simulink model "s_b16a4x32kf"  (R2018a)
settings: Solver=VariableStepDiscrete  StartTime=0.0  StopTime=1000  RelTol=1e-3
undefined symbols (not defined in the file): fft_stages, n_bits_ants, n_bits_xengs
libraries: xbsIndex_r4 x23740, casper_library_misc x48, casper_library_delays x8, xps_library x4, casper_library_scopes x1
(part 126 of 219)

== system s_b16a4x32kf/sys3/xeng/baseline_tap2/dual_pol_cmac/cmac ==
  a+bi : Inport
  c+di : Inport  Port=2
  acc_in : Inport  Port=3
  sync : Inport  Port=4
  valid_in : Inport  Port=5
  Constant1 : xbsIndex_r4/Constant  const=0  gui_display_data_type=Fixed-point  arith_type=Unsigned  n_bits=bit_growth  bin_pt=0  preci_type=Single  exp_width=8  frac_width=24  explicit_period=on  period=1  equ=P=C  opselect=C  inp2=PCIN>>17  opr=+  inp1=P  carry=CIN  dbl_ovrd=off  block_type=constant
      settings: block_version=9.2.01
  Constant2 : xbsIndex_r4/Constant  const=0  gui_display_data_type=Fixed-point  arith_type=Unsigned  n_bits=1  bin_pt=0  preci_type=Single  exp_width=8  frac_width=24  explicit_period=off  period=1  equ=P=C  opselect=C  inp2=PCIN>>17  opr=+  inp1=P  carry=CIN  dbl_ovrd=off  block_type=constant
      settings: block_version=9.2.01
  Counter : xbsIndex_r4/Counter  cnt_type=Count Limited  cnt_to=acc_len - 1  operation=Up  start_count=0  cnt_by_val=1  arith_type=Unsigned  n_bits=bit_growth  bin_pt=0  load_pin=off  rst=on  en=off  explicit_period=off  period=1  use_behavioral_HDL=off  implementation=Fabric  use_rpm=on  dbl_ovrd=off  block_type=counter
      settings: xl_area=[0, 0, 0, 0, 0, 0, 0]  block_version=9.2.01
  Delay : xbsIndex_r4/Delay  rst=off  infoeditControl=Selection of Reset will increase slice count due to use of real FFs and instead of SRLs  en=off  latency=add_latency + mult_latency - 1  reg_retiming=on  dbl_ovrd=off  block_type=delay
      settings: xl_area=[0, 0, 0, 0, 0, 0, 0]  block_version=9.2.01
  Relational : xbsIndex_r4/Relational  mode=a=b  op_type=Bool  en=off  latency=1  dbl_ovrd=off  block_type=relational
      settings: xl_area=[0, 0, 0, 0, 0, 0, 0]  block_version=9.2.01
  Terminator : Terminator
  acc : Subsystem
  acc1 : Subsystem
  c_to_ri1 : Subsystem
  c_to_ri2 : Subsystem
  cmult* : Subsystem  AncestorBlock=casper_library_multipliers/cmult  mask(cmult){n_bits_a=8, bin_pt_a=7, n_bits_b=8, bin_pt_b=7, n_bits_ab=25, bin_pt_ab=14, quantization=Truncate, overflow=Wrap, in_latency=0, mult_latency=4, add_latency=3, conv_latency=0, conjugated=on, async=off, pipelined_enable=on, multiplier_implementation=embedded multiplier core}
      mask prompts: n_bits_a "Number of Bits 'a'"; bin_pt_a "Binary Point 'a'"; n_bits_b "Number of Bits 'b'"; bin_pt_b "Binary Point 'b'"; n_bits_ab "Number of Bits 'ab'"; bin_pt_ab "Binary Point 'ab'"; in_latency "Input latency"; mult_latency "Multiplier Latency"; add_latency "Adder Latency"; conv_latency "Convert latency"; conjugated "Conjugate"; async "asynchronous operation"; pipelined_enable "enable pipeline"; multiplier_implementation "Multiplier implementation"
      mask help:
      | Multiplies two complex numbers using 4 multipliers and 2 adders.
      | Conjugation is optional.
      mask init: same as s_b16a4x32kf/sys0/xeng/auto_tap/dual_pol_cmac/cmac/cmult*
      settings: AttributesFormatString=|
      | 8_7 * 8_7 ==> 25_14
      | Truncate, Wrap
      | Latency=0
      mask TypeOptions quantization: Truncate | Round  (unbiased: +/- Inf) | Round  (unbiased: Even Values)
      mask TypeOptions overflow: Wrap | Saturate | Flag as error
      mask TypeOptions multiplier_implementation: behavioral HDL | standard core | embedded multiplier core
  ri_to_c : Subsystem
  acc_out : Outport
  valid_out : Outport  Port=2
  wires:
  cmult*/1(ab) -> c_to_ri1/1(In1)
  valid_in/1 -> acc1/4(valid_in)
  acc1/2(valid_out) -> valid_out/1
  acc/2(valid_out) -> Terminator/1
  Constant2/1 -> acc/4(valid_in)
  Delay/1 -> Counter/1
  sync/1 -> Delay/1
  Constant1/1 -> Relational/2
  Counter/1 -> Relational/1
  Relational/1 -> acc1/1(rst), acc/1(rst)
  c_to_ri2/2(Out2) -> acc1/3(acc_in)
  ri_to_c/1(Out1) -> acc_out/1
  acc1/1(acc_out) -> ri_to_c/2(In2)
  acc_in/1 -> c_to_ri2/1(In1)
  c+di/1 -> cmult*/2(b)
  a+bi/1 -> cmult*/1(a)
  c_to_ri1/1(Out1) -> acc/2(din)  "auto_real"
  c_to_ri1/2(Out2) -> acc1/2(din)
  acc/1(acc_out) -> ri_to_c/1(In1)
  c_to_ri2/1(Out1) -> acc/3(acc_in)

== system s_b16a4x32kf/sys3/xeng/baseline_tap2/dual_pol_cmac/cmac1 ==
  a+bi : Inport
  c+di : Inport  Port=2
  acc_in : Inport  Port=3
  sync : Inport  Port=4
  valid_in : Inport  Port=5
  Constant1 : xbsIndex_r4/Constant  const=0  gui_display_data_type=Fixed-point  arith_type=Unsigned  n_bits=bit_growth  bin_pt=0  preci_type=Single  exp_width=8  frac_width=24  explicit_period=on  period=1  equ=P=C  opselect=C  inp2=PCIN>>17  opr=+  inp1=P  carry=CIN  dbl_ovrd=off  block_type=constant
      settings: block_version=9.2.01
  Constant2 : xbsIndex_r4/Constant  const=0  gui_display_data_type=Fixed-point  arith_type=Unsigned  n_bits=1  bin_pt=0  preci_type=Single  exp_width=8  frac_width=24  explicit_period=off  period=1  equ=P=C  opselect=C  inp2=PCIN>>17  opr=+  inp1=P  carry=CIN  dbl_ovrd=off  block_type=constant
      settings: block_version=9.2.01
  Counter : xbsIndex_r4/Counter  cnt_type=Count Limited  cnt_to=acc_len - 1  operation=Up  start_count=0  cnt_by_val=1  arith_type=Unsigned  n_bits=bit_growth  bin_pt=0  load_pin=off  rst=on  en=off  explicit_period=off  period=1  use_behavioral_HDL=off  implementation=Fabric  use_rpm=on  dbl_ovrd=off  block_type=counter
      settings: xl_area=[0, 0, 0, 0, 0, 0, 0]  block_version=9.2.01
  Delay : xbsIndex_r4/Delay  rst=off  infoeditControl=Selection of Reset will increase slice count due to use of real FFs and instead of SRLs  en=off  latency=add_latency + mult_latency - 1  reg_retiming=on  dbl_ovrd=off  block_type=delay
      settings: xl_area=[0, 0, 0, 0, 0, 0, 0]  block_version=9.2.01
  Relational : xbsIndex_r4/Relational  mode=a=b  op_type=Bool  en=off  latency=1  dbl_ovrd=off  block_type=relational
      settings: xl_area=[0, 0, 0, 0, 0, 0, 0]  block_version=9.2.01
  Terminator : Terminator
  acc : Subsystem
  acc1 : Subsystem
  c_to_ri1 : Subsystem
  c_to_ri2 : Subsystem
  cmult* : Subsystem  AncestorBlock=casper_library_multipliers/cmult  mask(cmult){n_bits_a=8, bin_pt_a=7, n_bits_b=8, bin_pt_b=7, n_bits_ab=25, bin_pt_ab=14, quantization=Truncate, overflow=Wrap, in_latency=0, mult_latency=4, add_latency=3, conv_latency=0, conjugated=on, async=off, pipelined_enable=on, multiplier_implementation=embedded multiplier core}
      mask prompts: n_bits_a "Number of Bits 'a'"; bin_pt_a "Binary Point 'a'"; n_bits_b "Number of Bits 'b'"; bin_pt_b "Binary Point 'b'"; n_bits_ab "Number of Bits 'ab'"; bin_pt_ab "Binary Point 'ab'"; in_latency "Input latency"; mult_latency "Multiplier Latency"; add_latency "Adder Latency"; conv_latency "Convert latency"; conjugated "Conjugate"; async "asynchronous operation"; pipelined_enable "enable pipeline"; multiplier_implementation "Multiplier implementation"
      mask help:
      | Multiplies two complex numbers using 4 multipliers and 2 adders.
      | Conjugation is optional.
      mask init: same as s_b16a4x32kf/sys0/xeng/auto_tap/dual_pol_cmac/cmac/cmult*
      settings: AttributesFormatString=|
      | 8_7 * 8_7 ==> 25_14
      | Truncate, Wrap
      | Latency=0
      mask TypeOptions quantization: Truncate | Round  (unbiased: +/- Inf) | Round  (unbiased: Even Values)
      mask TypeOptions overflow: Wrap | Saturate | Flag as error
      mask TypeOptions multiplier_implementation: behavioral HDL | standard core | embedded multiplier core
  ri_to_c : Subsystem
  acc_out : Outport
  valid_out : Outport  Port=2
  wires:
  cmult*/1(ab) -> c_to_ri1/1(In1)
  valid_in/1 -> acc1/4(valid_in)
  acc1/2(valid_out) -> valid_out/1
  acc/2(valid_out) -> Terminator/1
  Constant2/1 -> acc/4(valid_in)
  Delay/1 -> Counter/1
  sync/1 -> Delay/1
  Constant1/1 -> Relational/2
  Counter/1 -> Relational/1
  Relational/1 -> acc1/1(rst), acc/1(rst)
  c_to_ri2/2(Out2) -> acc1/3(acc_in)
  ri_to_c/1(Out1) -> acc_out/1
  acc1/1(acc_out) -> ri_to_c/2(In2)
  acc_in/1 -> c_to_ri2/1(In1)
  c+di/1 -> cmult*/2(b)
  a+bi/1 -> cmult*/1(a)
  c_to_ri1/1(Out1) -> acc/2(din)  "auto_real"
  c_to_ri1/2(Out2) -> acc1/2(din)
  acc/1(acc_out) -> ri_to_c/1(In1)
  c_to_ri2/1(Out1) -> acc/3(acc_in)

== system s_b16a4x32kf/sys3/xeng/baseline_tap2/dual_pol_cmac/cmac2 ==
  a+bi : Inport
  c+di : Inport  Port=2
  acc_in : Inport  Port=3
  sync : Inport  Port=4
  valid_in : Inport  Port=5
  Constant1 : xbsIndex_r4/Constant  const=0  gui_display_data_type=Fixed-point  arith_type=Unsigned  n_bits=bit_growth  bin_pt=0  preci_type=Single  exp_width=8  frac_width=24  explicit_period=on  period=1  equ=P=C  opselect=C  inp2=PCIN>>17  opr=+  inp1=P  carry=CIN  dbl_ovrd=off  block_type=constant
      settings: block_version=9.2.01
  Constant2 : xbsIndex_r4/Constant  const=0  gui_display_data_type=Fixed-point  arith_type=Unsigned  n_bits=1  bin_pt=0  preci_type=Single  exp_width=8  frac_width=24  explicit_period=off  period=1  equ=P=C  opselect=C  inp2=PCIN>>17  opr=+  inp1=P  carry=CIN  dbl_ovrd=off  block_type=constant
      settings: block_version=9.2.01
  Counter : xbsIndex_r4/Counter  cnt_type=Count Limited  cnt_to=acc_len - 1  operation=Up  start_count=0  cnt_by_val=1  arith_type=Unsigned  n_bits=bit_growth  bin_pt=0  load_pin=off  rst=on  en=off  explicit_period=off  period=1  use_behavioral_HDL=off  implementation=Fabric  use_rpm=on  dbl_ovrd=off  block_type=counter
      settings: xl_area=[0, 0, 0, 0, 0, 0, 0]  block_version=9.2.01
  Delay : xbsIndex_r4/Delay  rst=off  infoeditControl=Selection of Reset will increase slice count due to use of real FFs and instead of SRLs  en=off  latency=add_latency + mult_latency - 1  reg_retiming=on  dbl_ovrd=off  block_type=delay
      settings: xl_area=[0, 0, 0, 0, 0, 0, 0]  block_version=9.2.01
  Relational : xbsIndex_r4/Relational  mode=a=b  op_type=Bool  en=off  latency=1  dbl_ovrd=off  block_type=relational
      settings: xl_area=[0, 0, 0, 0, 0, 0, 0]  block_version=9.2.01
  Terminator : Terminator
  acc : Subsystem
  acc1 : Subsystem
  c_to_ri1 : Subsystem
  c_to_ri2 : Subsystem
  cmult* : Subsystem  AncestorBlock=casper_library_multipliers/cmult  mask(cmult){n_bits_a=8, bin_pt_a=7, n_bits_b=8, bin_pt_b=7, n_bits_ab=25, bin_pt_ab=14, quantization=Truncate, overflow=Wrap, in_latency=0, mult_latency=4, add_latency=3, conv_latency=0, conjugated=on, async=off, pipelined_enable=on, multiplier_implementation=embedded multiplier core}
      mask prompts: n_bits_a "Number of Bits 'a'"; bin_pt_a "Binary Point 'a'"; n_bits_b "Number of Bits 'b'"; bin_pt_b "Binary Point 'b'"; n_bits_ab "Number of Bits 'ab'"; bin_pt_ab "Binary Point 'ab'"; in_latency "Input latency"; mult_latency "Multiplier Latency"; add_latency "Adder Latency"; conv_latency "Convert latency"; conjugated "Conjugate"; async "asynchronous operation"; pipelined_enable "enable pipeline"; multiplier_implementation "Multiplier implementation"
      mask help:
      | Multiplies two complex numbers using 4 multipliers and 2 adders.
      | Conjugation is optional.
      mask init: same as s_b16a4x32kf/sys0/xeng/auto_tap/dual_pol_cmac/cmac/cmult*
      settings: AttributesFormatString=|
      | 8_7 * 8_7 ==> 25_14
      | Truncate, Wrap
      | Latency=0
      mask TypeOptions quantization: Truncate | Round  (unbiased: +/- Inf) | Round  (unbiased: Even Values)
      mask TypeOptions overflow: Wrap | Saturate | Flag as error
      mask TypeOptions multiplier_implementation: behavioral HDL | standard core | embedded multiplier core
  ri_to_c : Subsystem
  acc_out : Outport
  valid_out : Outport  Port=2
  wires:
  cmult*/1(ab) -> c_to_ri1/1(In1)
  valid_in/1 -> acc1/4(valid_in)
  acc1/2(valid_out) -> valid_out/1
  acc/2(valid_out) -> Terminator/1
  Constant2/1 -> acc/4(valid_in)
  Delay/1 -> Counter/1
  sync/1 -> Delay/1
  Constant1/1 -> Relational/2
  Counter/1 -> Relational/1
  Relational/1 -> acc1/1(rst), acc/1(rst)
  c_to_ri2/2(Out2) -> acc1/3(acc_in)
  ri_to_c/1(Out1) -> acc_out/1
  acc1/1(acc_out) -> ri_to_c/2(In2)
  acc_in/1 -> c_to_ri2/1(In1)
  c+di/1 -> cmult*/2(b)
  a+bi/1 -> cmult*/1(a)
  c_to_ri1/1(Out1) -> acc/2(din)  "auto_real"
  c_to_ri1/2(Out2) -> acc1/2(din)
  acc/1(acc_out) -> ri_to_c/1(In1)
  c_to_ri2/1(Out1) -> acc/3(acc_in)

== system s_b16a4x32kf/sys3/xeng/baseline_tap2/dual_pol_cmac/cmac3 ==
  a+bi : Inport
  c+di : Inport  Port=2
  acc_in : Inport  Port=3
  sync : Inport  Port=4
  valid_in : Inport  Port=5
  Constant1 : xbsIndex_r4/Constant  const=0  gui_display_data_type=Fixed-point  arith_type=Unsigned  n_bits=bit_growth  bin_pt=0  preci_type=Single  exp_width=8  frac_width=24  explicit_period=on  period=1  equ=P=C  opselect=C  inp2=PCIN>>17  opr=+  inp1=P  carry=CIN  dbl_ovrd=off  block_type=constant
      settings: block_version=9.2.01
  Constant2 : xbsIndex_r4/Constant  const=0  gui_display_data_type=Fixed-point  arith_type=Unsigned  n_bits=1  bin_pt=0  preci_type=Single  exp_width=8  frac_width=24  explicit_period=off  period=1  equ=P=C  opselect=C  inp2=PCIN>>17  opr=+  inp1=P  carry=CIN  dbl_ovrd=off  block_type=constant
      settings: block_version=9.2.01
  Counter : xbsIndex_r4/Counter  cnt_type=Count Limited  cnt_to=acc_len - 1  operation=Up  start_count=0  cnt_by_val=1  arith_type=Unsigned  n_bits=bit_growth  bin_pt=0  load_pin=off  rst=on  en=off  explicit_period=off  period=1  use_behavioral_HDL=off  implementation=Fabric  use_rpm=on  dbl_ovrd=off  block_type=counter
      settings: xl_area=[0, 0, 0, 0, 0, 0, 0]  block_version=9.2.01
  Delay : xbsIndex_r4/Delay  rst=off  infoeditControl=Selection of Reset will increase slice count due to use of real FFs and instead of SRLs  en=off  latency=add_latency + mult_latency - 1  reg_retiming=on  dbl_ovrd=off  block_type=delay
      settings: xl_area=[0, 0, 0, 0, 0, 0, 0]  block_version=9.2.01
  Relational : xbsIndex_r4/Relational  mode=a=b  op_type=Bool  en=off  latency=1  dbl_ovrd=off  block_type=relational
      settings: xl_area=[0, 0, 0, 0, 0, 0, 0]  block_version=9.2.01
  Terminator : Terminator
  acc : Subsystem
  acc1 : Subsystem
  c_to_ri1 : Subsystem
  c_to_ri2 : Subsystem
  cmult* : Subsystem  AncestorBlock=casper_library_multipliers/cmult  mask(cmult){n_bits_a=8, bin_pt_a=7, n_bits_b=8, bin_pt_b=7, n_bits_ab=25, bin_pt_ab=14, quantization=Truncate, overflow=Wrap, in_latency=0, mult_latency=4, add_latency=3, conv_latency=0, conjugated=on, async=off, pipelined_enable=on, multiplier_implementation=embedded multiplier core}
      mask prompts: n_bits_a "Number of Bits 'a'"; bin_pt_a "Binary Point 'a'"; n_bits_b "Number of Bits 'b'"; bin_pt_b "Binary Point 'b'"; n_bits_ab "Number of Bits 'ab'"; bin_pt_ab "Binary Point 'ab'"; in_latency "Input latency"; mult_latency "Multiplier Latency"; add_latency "Adder Latency"; conv_latency "Convert latency"; conjugated "Conjugate"; async "asynchronous operation"; pipelined_enable "enable pipeline"; multiplier_implementation "Multiplier implementation"
      mask help:
      | Multiplies two complex numbers using 4 multipliers and 2 adders.
      | Conjugation is optional.
      mask init: same as s_b16a4x32kf/sys0/xeng/auto_tap/dual_pol_cmac/cmac/cmult*
      settings: AttributesFormatString=|
      | 8_7 * 8_7 ==> 25_14
      | Truncate, Wrap
      | Latency=0
      mask TypeOptions quantization: Truncate | Round  (unbiased: +/- Inf) | Round  (unbiased: Even Values)
      mask TypeOptions overflow: Wrap | Saturate | Flag as error
      mask TypeOptions multiplier_implementation: behavioral HDL | standard core | embedded multiplier core
  ri_to_c : Subsystem
  acc_out : Outport
  valid_out : Outport  Port=2
  wires:
  cmult*/1(ab) -> c_to_ri1/1(In1)
  valid_in/1 -> acc1/4(valid_in)
  acc1/2(valid_out) -> valid_out/1
  acc/2(valid_out) -> Terminator/1
  Constant2/1 -> acc/4(valid_in)
  Delay/1 -> Counter/1
  sync/1 -> Delay/1
  Constant1/1 -> Relational/2
  Counter/1 -> Relational/1
  Relational/1 -> acc1/1(rst), acc/1(rst)
  c_to_ri2/2(Out2) -> acc1/3(acc_in)
  ri_to_c/1(Out1) -> acc_out/1
  acc1/1(acc_out) -> ri_to_c/2(In2)
  acc_in/1 -> c_to_ri2/1(In1)
  c+di/1 -> cmult*/2(b)
  a+bi/1 -> cmult*/1(a)
  c_to_ri1/1(Out1) -> acc/2(din)  "auto_real"
  c_to_ri1/2(Out2) -> acc1/2(din)
  acc/1(acc_out) -> ri_to_c/1(In1)
  c_to_ri2/1(Out1) -> acc/3(acc_in)

== system s_b16a4x32kf/sys3/xeng/baseline_tap3/dual_pol_cmac/cmac ==
  a+bi : Inport
  c+di : Inport  Port=2
  acc_in : Inport  Port=3
  sync : Inport  Port=4
  valid_in : Inport  Port=5
  Constant1 : xbsIndex_r4/Constant  const=0  gui_display_data_type=Fixed-point  arith_type=Unsigned  n_bits=bit_growth  bin_pt=0  preci_type=Single  exp_width=8  frac_width=24  explicit_period=on  period=1  equ=P=C  opselect=C  inp2=PCIN>>17  opr=+  inp1=P  carry=CIN  dbl_ovrd=off  block_type=constant
      settings: block_version=9.2.01
  Constant2 : xbsIndex_r4/Constant  const=0  gui_display_data_type=Fixed-point  arith_type=Unsigned  n_bits=1  bin_pt=0  preci_type=Single  exp_width=8  frac_width=24  explicit_period=off  period=1  equ=P=C  opselect=C  inp2=PCIN>>17  opr=+  inp1=P  carry=CIN  dbl_ovrd=off  block_type=constant
      settings: block_version=9.2.01
  Counter : xbsIndex_r4/Counter  cnt_type=Count Limited  cnt_to=acc_len - 1  operation=Up  start_count=0  cnt_by_val=1  arith_type=Unsigned  n_bits=bit_growth  bin_pt=0  load_pin=off  rst=on  en=off  explicit_period=off  period=1  use_behavioral_HDL=off  implementation=Fabric  use_rpm=on  dbl_ovrd=off  block_type=counter
      settings: xl_area=[0, 0, 0, 0, 0, 0, 0]  block_version=9.2.01
  Delay : xbsIndex_r4/Delay  rst=off  infoeditControl=Selection of Reset will increase slice count due to use of real FFs and instead of SRLs  en=off  latency=add_latency + mult_latency - 1  reg_retiming=on  dbl_ovrd=off  block_type=delay
      settings: xl_area=[0, 0, 0, 0, 0, 0, 0]  block_version=9.2.01
  Relational : xbsIndex_r4/Relational  mode=a=b  op_type=Bool  en=off  latency=1  dbl_ovrd=off  block_type=relational
      settings: xl_area=[0, 0, 0, 0, 0, 0, 0]  block_version=9.2.01
  Terminator : Terminator
  acc : Subsystem
  acc1 : Subsystem
  c_to_ri1 : Subsystem
  c_to_ri2 : Subsystem
  cmult* : Subsystem  AncestorBlock=casper_library_multipliers/cmult  mask(cmult){n_bits_a=8, bin_pt_a=7, n_bits_b=8, bin_pt_b=7, n_bits_ab=25, bin_pt_ab=14, quantization=Truncate, overflow=Wrap, in_latency=0, mult_latency=4, add_latency=3, conv_latency=0, conjugated=on, async=off, pipelined_enable=on, multiplier_implementation=embedded multiplier core}
      mask prompts: n_bits_a "Number of Bits 'a'"; bin_pt_a "Binary Point 'a'"; n_bits_b "Number of Bits 'b'"; bin_pt_b "Binary Point 'b'"; n_bits_ab "Number of Bits 'ab'"; bin_pt_ab "Binary Point 'ab'"; in_latency "Input latency"; mult_latency "Multiplier Latency"; add_latency "Adder Latency"; conv_latency "Convert latency"; conjugated "Conjugate"; async "asynchronous operation"; pipelined_enable "enable pipeline"; multiplier_implementation "Multiplier implementation"
      mask help:
      | Multiplies two complex numbers using 4 multipliers and 2 adders.
      | Conjugation is optional.
      mask init: same as s_b16a4x32kf/sys0/xeng/auto_tap/dual_pol_cmac/cmac/cmult*
      settings: AttributesFormatString=|
      | 8_7 * 8_7 ==> 25_14
      | Truncate, Wrap
      | Latency=0
      mask TypeOptions quantization: Truncate | Round  (unbiased: +/- Inf) | Round  (unbiased: Even Values)
      mask TypeOptions overflow: Wrap | Saturate | Flag as error
      mask TypeOptions multiplier_implementation: behavioral HDL | standard core | embedded multiplier core
  ri_to_c : Subsystem
  acc_out : Outport
  valid_out : Outport  Port=2
  wires:
  cmult*/1(ab) -> c_to_ri1/1(In1)
  valid_in/1 -> acc1/4(valid_in)
  acc1/2(valid_out) -> valid_out/1
  acc/2(valid_out) -> Terminator/1
  Constant2/1 -> acc/4(valid_in)
  Delay/1 -> Counter/1
  sync/1 -> Delay/1
  Constant1/1 -> Relational/2
  Counter/1 -> Relational/1
  Relational/1 -> acc1/1(rst), acc/1(rst)
  c_to_ri2/2(Out2) -> acc1/3(acc_in)
  ri_to_c/1(Out1) -> acc_out/1
  acc1/1(acc_out) -> ri_to_c/2(In2)
  acc_in/1 -> c_to_ri2/1(In1)
  c+di/1 -> cmult*/2(b)
  a+bi/1 -> cmult*/1(a)
  c_to_ri1/1(Out1) -> acc/2(din)  "auto_real"
  c_to_ri1/2(Out2) -> acc1/2(din)
  acc/1(acc_out) -> ri_to_c/1(In1)
  c_to_ri2/1(Out1) -> acc/3(acc_in)

== system s_b16a4x32kf/sys3/xeng/baseline_tap3/dual_pol_cmac/cmac1 ==
  a+bi : Inport
  c+di : Inport  Port=2
  acc_in : Inport  Port=3
  sync : Inport  Port=4
  valid_in : Inport  Port=5
  Constant1 : xbsIndex_r4/Constant  const=0  gui_display_data_type=Fixed-point  arith_type=Unsigned  n_bits=bit_growth  bin_pt=0  preci_type=Single  exp_width=8  frac_width=24  explicit_period=on  period=1  equ=P=C  opselect=C  inp2=PCIN>>17  opr=+  inp1=P  carry=CIN  dbl_ovrd=off  block_type=constant
      settings: block_version=9.2.01
  Constant2 : xbsIndex_r4/Constant  const=0  gui_display_data_type=Fixed-point  arith_type=Unsigned  n_bits=1  bin_pt=0  preci_type=Single  exp_width=8  frac_width=24  explicit_period=off  period=1  equ=P=C  opselect=C  inp2=PCIN>>17  opr=+  inp1=P  carry=CIN  dbl_ovrd=off  block_type=constant
      settings: block_version=9.2.01
  Counter : xbsIndex_r4/Counter  cnt_type=Count Limited  cnt_to=acc_len - 1  operation=Up  start_count=0  cnt_by_val=1  arith_type=Unsigned  n_bits=bit_growth  bin_pt=0  load_pin=off  rst=on  en=off  explicit_period=off  period=1  use_behavioral_HDL=off  implementation=Fabric  use_rpm=on  dbl_ovrd=off  block_type=counter
      settings: xl_area=[0, 0, 0, 0, 0, 0, 0]  block_version=9.2.01
  Delay : xbsIndex_r4/Delay  rst=off  infoeditControl=Selection of Reset will increase slice count due to use of real FFs and instead of SRLs  en=off  latency=add_latency + mult_latency - 1  reg_retiming=on  dbl_ovrd=off  block_type=delay
      settings: xl_area=[0, 0, 0, 0, 0, 0, 0]  block_version=9.2.01
  Relational : xbsIndex_r4/Relational  mode=a=b  op_type=Bool  en=off  latency=1  dbl_ovrd=off  block_type=relational
      settings: xl_area=[0, 0, 0, 0, 0, 0, 0]  block_version=9.2.01
  Terminator : Terminator
  acc : Subsystem
  acc1 : Subsystem
  c_to_ri1 : Subsystem
  c_to_ri2 : Subsystem
  cmult* : Subsystem  AncestorBlock=casper_library_multipliers/cmult  mask(cmult){n_bits_a=8, bin_pt_a=7, n_bits_b=8, bin_pt_b=7, n_bits_ab=25, bin_pt_ab=14, quantization=Truncate, overflow=Wrap, in_latency=0, mult_latency=4, add_latency=3, conv_latency=0, conjugated=on, async=off, pipelined_enable=on, multiplier_implementation=embedded multiplier core}
      mask prompts: n_bits_a "Number of Bits 'a'"; bin_pt_a "Binary Point 'a'"; n_bits_b "Number of Bits 'b'"; bin_pt_b "Binary Point 'b'"; n_bits_ab "Number of Bits 'ab'"; bin_pt_ab "Binary Point 'ab'"; in_latency "Input latency"; mult_latency "Multiplier Latency"; add_latency "Adder Latency"; conv_latency "Convert latency"; conjugated "Conjugate"; async "asynchronous operation"; pipelined_enable "enable pipeline"; multiplier_implementation "Multiplier implementation"
      mask help:
      | Multiplies two complex numbers using 4 multipliers and 2 adders.
      | Conjugation is optional.
      mask init: same as s_b16a4x32kf/sys0/xeng/auto_tap/dual_pol_cmac/cmac/cmult*
      settings: AttributesFormatString=|
      | 8_7 * 8_7 ==> 25_14
      | Truncate, Wrap
      | Latency=0
      mask TypeOptions quantization: Truncate | Round  (unbiased: +/- Inf) | Round  (unbiased: Even Values)
      mask TypeOptions overflow: Wrap | Saturate | Flag as error
      mask TypeOptions multiplier_implementation: behavioral HDL | standard core | embedded multiplier core
  ri_to_c : Subsystem
  acc_out : Outport
  valid_out : Outport  Port=2
  wires:
  cmult*/1(ab) -> c_to_ri1/1(In1)
  valid_in/1 -> acc1/4(valid_in)
  acc1/2(valid_out) -> valid_out/1
  acc/2(valid_out) -> Terminator/1
  Constant2/1 -> acc/4(valid_in)
  Delay/1 -> Counter/1
  sync/1 -> Delay/1
  Constant1/1 -> Relational/2
  Counter/1 -> Relational/1
  Relational/1 -> acc1/1(rst), acc/1(rst)
  c_to_ri2/2(Out2) -> acc1/3(acc_in)
  ri_to_c/1(Out1) -> acc_out/1
  acc1/1(acc_out) -> ri_to_c/2(In2)
  acc_in/1 -> c_to_ri2/1(In1)
  c+di/1 -> cmult*/2(b)
  a+bi/1 -> cmult*/1(a)
  c_to_ri1/1(Out1) -> acc/2(din)  "auto_real"
  c_to_ri1/2(Out2) -> acc1/2(din)
  acc/1(acc_out) -> ri_to_c/1(In1)
  c_to_ri2/1(Out1) -> acc/3(acc_in)

== system s_b16a4x32kf/sys3/xeng/baseline_tap3/dual_pol_cmac/cmac2 ==
  a+bi : Inport
  c+di : Inport  Port=2
  acc_in : Inport  Port=3
  sync : Inport  Port=4
  valid_in : Inport  Port=5
  Constant1 : xbsIndex_r4/Constant  const=0  gui_display_data_type=Fixed-point  arith_type=Unsigned  n_bits=bit_growth  bin_pt=0  preci_type=Single  exp_width=8  frac_width=24  explicit_period=on  period=1  equ=P=C  opselect=C  inp2=PCIN>>17  opr=+  inp1=P  carry=CIN  dbl_ovrd=off  block_type=constant
      settings: block_version=9.2.01
  Constant2 : xbsIndex_r4/Constant  const=0  gui_display_data_type=Fixed-point  arith_type=Unsigned  n_bits=1  bin_pt=0  preci_type=Single  exp_width=8  frac_width=24  explicit_period=off  period=1  equ=P=C  opselect=C  inp2=PCIN>>17  opr=+  inp1=P  carry=CIN  dbl_ovrd=off  block_type=constant
      settings: block_version=9.2.01
  Counter : xbsIndex_r4/Counter  cnt_type=Count Limited  cnt_to=acc_len - 1  operation=Up  start_count=0  cnt_by_val=1  arith_type=Unsigned  n_bits=bit_growth  bin_pt=0  load_pin=off  rst=on  en=off  explicit_period=off  period=1  use_behavioral_HDL=off  implementation=Fabric  use_rpm=on  dbl_ovrd=off  block_type=counter
      settings: xl_area=[0, 0, 0, 0, 0, 0, 0]  block_version=9.2.01
  Delay : xbsIndex_r4/Delay  rst=off  infoeditControl=Selection of Reset will increase slice count due to use of real FFs and instead of SRLs  en=off  latency=add_latency + mult_latency - 1  reg_retiming=on  dbl_ovrd=off  block_type=delay
      settings: xl_area=[0, 0, 0, 0, 0, 0, 0]  block_version=9.2.01
  Relational : xbsIndex_r4/Relational  mode=a=b  op_type=Bool  en=off  latency=1  dbl_ovrd=off  block_type=relational
      settings: xl_area=[0, 0, 0, 0, 0, 0, 0]  block_version=9.2.01
  Terminator : Terminator
  acc : Subsystem
  acc1 : Subsystem
  c_to_ri1 : Subsystem
  c_to_ri2 : Subsystem
  cmult* : Subsystem  AncestorBlock=casper_library_multipliers/cmult  mask(cmult){n_bits_a=8, bin_pt_a=7, n_bits_b=8, bin_pt_b=7, n_bits_ab=25, bin_pt_ab=14, quantization=Truncate, overflow=Wrap, in_latency=0, mult_latency=4, add_latency=3, conv_latency=0, conjugated=on, async=off, pipelined_enable=on, multiplier_implementation=embedded multiplier core}
      mask prompts: n_bits_a "Number of Bits 'a'"; bin_pt_a "Binary Point 'a'"; n_bits_b "Number of Bits 'b'"; bin_pt_b "Binary Point 'b'"; n_bits_ab "Number of Bits 'ab'"; bin_pt_ab "Binary Point 'ab'"; in_latency "Input latency"; mult_latency "Multiplier Latency"; add_latency "Adder Latency"; conv_latency "Convert latency"; conjugated "Conjugate"; async "asynchronous operation"; pipelined_enable "enable pipeline"; multiplier_implementation "Multiplier implementation"
      mask help:
      | Multiplies two complex numbers using 4 multipliers and 2 adders.
      | Conjugation is optional.
      mask init: same as s_b16a4x32kf/sys0/xeng/auto_tap/dual_pol_cmac/cmac/cmult*
      settings: AttributesFormatString=|
      | 8_7 * 8_7 ==> 25_14
      | Truncate, Wrap
      | Latency=0
      mask TypeOptions quantization: Truncate | Round  (unbiased: +/- Inf) | Round  (unbiased: Even Values)
      mask TypeOptions overflow: Wrap | Saturate | Flag as error
      mask TypeOptions multiplier_implementation: behavioral HDL | standard core | embedded multiplier core
  ri_to_c : Subsystem
  acc_out : Outport
  valid_out : Outport  Port=2
  wires:
  cmult*/1(ab) -> c_to_ri1/1(In1)
  valid_in/1 -> acc1/4(valid_in)
  acc1/2(valid_out) -> valid_out/1
  acc/2(valid_out) -> Terminator/1
  Constant2/1 -> acc/4(valid_in)
  Delay/1 -> Counter/1
  sync/1 -> Delay/1
  Constant1/1 -> Relational/2
  Counter/1 -> Relational/1
  Relational/1 -> acc1/1(rst), acc/1(rst)
  c_to_ri2/2(Out2) -> acc1/3(acc_in)
  ri_to_c/1(Out1) -> acc_out/1
  acc1/1(acc_out) -> ri_to_c/2(In2)
  acc_in/1 -> c_to_ri2/1(In1)
  c+di/1 -> cmult*/2(b)
  a+bi/1 -> cmult*/1(a)
  c_to_ri1/1(Out1) -> acc/2(din)  "auto_real"
  c_to_ri1/2(Out2) -> acc1/2(din)
  acc/1(acc_out) -> ri_to_c/1(In1)
  c_to_ri2/1(Out1) -> acc/3(acc_in)

== system s_b16a4x32kf/sys3/xeng/baseline_tap3/dual_pol_cmac/cmac3 ==
  a+bi : Inport
  c+di : Inport  Port=2
  acc_in : Inport  Port=3
  sync : Inport  Port=4
  valid_in : Inport  Port=5
  Constant1 : xbsIndex_r4/Constant  const=0  gui_display_data_type=Fixed-point  arith_type=Unsigned  n_bits=bit_growth  bin_pt=0  preci_type=Single  exp_width=8  frac_width=24  explicit_period=on  period=1  equ=P=C  opselect=C  inp2=PCIN>>17  opr=+  inp1=P  carry=CIN  dbl_ovrd=off  block_type=constant
      settings: block_version=9.2.01
  Constant2 : xbsIndex_r4/Constant  const=0  gui_display_data_type=Fixed-point  arith_type=Unsigned  n_bits=1  bin_pt=0  preci_type=Single  exp_width=8  frac_width=24  explicit_period=off  period=1  equ=P=C  opselect=C  inp2=PCIN>>17  opr=+  inp1=P  carry=CIN  dbl_ovrd=off  block_type=constant
      settings: block_version=9.2.01
  Counter : xbsIndex_r4/Counter  cnt_type=Count Limited  cnt_to=acc_len - 1  operation=Up  start_count=0  cnt_by_val=1  arith_type=Unsigned  n_bits=bit_growth  bin_pt=0  load_pin=off  rst=on  en=off  explicit_period=off  period=1  use_behavioral_HDL=off  implementation=Fabric  use_rpm=on  dbl_ovrd=off  block_type=counter
      settings: xl_area=[0, 0, 0, 0, 0, 0, 0]  block_version=9.2.01
  Delay : xbsIndex_r4/Delay  rst=off  infoeditControl=Selection of Reset will increase slice count due to use of real FFs and instead of SRLs  en=off  latency=add_latency + mult_latency - 1  reg_retiming=on  dbl_ovrd=off  block_type=delay
      settings: xl_area=[0, 0, 0, 0, 0, 0, 0]  block_version=9.2.01
  Relational : xbsIndex_r4/Relational  mode=a=b  op_type=Bool  en=off  latency=1  dbl_ovrd=off  block_type=relational
      settings: xl_area=[0, 0, 0, 0, 0, 0, 0]  block_version=9.2.01
  Terminator : Terminator
  acc : Subsystem
  acc1 : Subsystem
  c_to_ri1 : Subsystem
  c_to_ri2 : Subsystem
  cmult* : Subsystem  AncestorBlock=casper_library_multipliers/cmult  mask(cmult){n_bits_a=8, bin_pt_a=7, n_bits_b=8, bin_pt_b=7, n_bits_ab=25, bin_pt_ab=14, quantization=Truncate, overflow=Wrap, in_latency=0, mult_latency=4, add_latency=3, conv_latency=0, conjugated=on, async=off, pipelined_enable=on, multiplier_implementation=embedded multiplier core}
      mask prompts: n_bits_a "Number of Bits 'a'"; bin_pt_a "Binary Point 'a'"; n_bits_b "Number of Bits 'b'"; bin_pt_b "Binary Point 'b'"; n_bits_ab "Number of Bits 'ab'"; bin_pt_ab "Binary Point 'ab'"; in_latency "Input latency"; mult_latency "Multiplier Latency"; add_latency "Adder Latency"; conv_latency "Convert latency"; conjugated "Conjugate"; async "asynchronous operation"; pipelined_enable "enable pipeline"; multiplier_implementation "Multiplier implementation"
      mask help:
      | Multiplies two complex numbers using 4 multipliers and 2 adders.
      | Conjugation is optional.
      mask init: same as s_b16a4x32kf/sys0/xeng/auto_tap/dual_pol_cmac/cmac/cmult*
      settings: AttributesFormatString=|
      | 8_7 * 8_7 ==> 25_14
      | Truncate, Wrap
      | Latency=0
      mask TypeOptions quantization: Truncate | Round  (unbiased: +/- Inf) | Round  (unbiased: Even Values)
      mask TypeOptions overflow: Wrap | Saturate | Flag as error
      mask TypeOptions multiplier_implementation: behavioral HDL | standard core | embedded multiplier core
  ri_to_c : Subsystem
  acc_out : Outport
  valid_out : Outport  Port=2
  wires:
  cmult*/1(ab) -> c_to_ri1/1(In1)
  valid_in/1 -> acc1/4(valid_in)
  acc1/2(valid_out) -> valid_out/1
  acc/2(valid_out) -> Terminator/1
  Constant2/1 -> acc/4(valid_in)
  Delay/1 -> Counter/1
  sync/1 -> Delay/1
  Constant1/1 -> Relational/2
  Counter/1 -> Relational/1
  Relational/1 -> acc1/1(rst), acc/1(rst)
  c_to_ri2/2(Out2) -> acc1/3(acc_in)
  ri_to_c/1(Out1) -> acc_out/1
  acc1/1(acc_out) -> ri_to_c/2(In2)
  acc_in/1 -> c_to_ri2/1(In1)
  c+di/1 -> cmult*/2(b)
  a+bi/1 -> cmult*/1(a)
  c_to_ri1/1(Out1) -> acc/2(din)  "auto_real"
  c_to_ri1/2(Out2) -> acc1/2(din)
  acc/1(acc_out) -> ri_to_c/1(In1)
  c_to_ri2/1(Out1) -> acc/3(acc_in)

== system s_b16a4x32kf/sys3/xeng/baseline_tap4/dual_pol_cmac/cmac ==
  a+bi : Inport
  c+di : Inport  Port=2
  acc_in : Inport  Port=3
  sync : Inport  Port=4
  valid_in : Inport  Port=5
  Constant1 : xbsIndex_r4/Constant  const=0  gui_display_data_type=Fixed-point  arith_type=Unsigned  n_bits=bit_growth  bin_pt=0  preci_type=Single  exp_width=8  frac_width=24  explicit_period=on  period=1  equ=P=C  opselect=C  inp2=PCIN>>17  opr=+  inp1=P  carry=CIN  dbl_ovrd=off  block_type=constant
      settings: block_version=9.2.01
  Constant2 : xbsIndex_r4/Constant  const=0  gui_display_data_type=Fixed-point  arith_type=Unsigned  n_bits=1  bin_pt=0  preci_type=Single  exp_width=8  frac_width=24  explicit_period=off  period=1  equ=P=C  opselect=C  inp2=PCIN>>17  opr=+  inp1=P  carry=CIN  dbl_ovrd=off  block_type=constant
      settings: block_version=9.2.01
  Counter : xbsIndex_r4/Counter  cnt_type=Count Limited  cnt_to=acc_len - 1  operation=Up  start_count=0  cnt_by_val=1  arith_type=Unsigned  n_bits=bit_growth  bin_pt=0  load_pin=off  rst=on  en=off  explicit_period=off  period=1  use_behavioral_HDL=off  implementation=Fabric  use_rpm=on  dbl_ovrd=off  block_type=counter
      settings: xl_area=[0, 0, 0, 0, 0, 0, 0]  block_version=9.2.01
  Delay : xbsIndex_r4/Delay  rst=off  infoeditControl=Selection of Reset will increase slice count due to use of real FFs and instead of SRLs  en=off  latency=add_latency + mult_latency - 1  reg_retiming=on  dbl_ovrd=off  block_type=delay
      settings: xl_area=[0, 0, 0, 0, 0, 0, 0]  block_version=9.2.01
  Relational : xbsIndex_r4/Relational  mode=a=b  op_type=Bool  en=off  latency=1  dbl_ovrd=off  block_type=relational
      settings: xl_area=[0, 0, 0, 0, 0, 0, 0]  block_version=9.2.01
  Terminator : Terminator
  acc : Subsystem
  acc1 : Subsystem
  c_to_ri1 : Subsystem
  c_to_ri2 : Subsystem
  cmult* : Subsystem  AncestorBlock=casper_library_multipliers/cmult  mask(cmult){n_bits_a=8, bin_pt_a=7, n_bits_b=8, bin_pt_b=7, n_bits_ab=25, bin_pt_ab=14, quantization=Truncate, overflow=Wrap, in_latency=0, mult_latency=4, add_latency=3, conv_latency=0, conjugated=on, async=off, pipelined_enable=on, multiplier_implementation=embedded multiplier core}
      mask prompts: n_bits_a "Number of Bits 'a'"; bin_pt_a "Binary Point 'a'"; n_bits_b "Number of Bits 'b'"; bin_pt_b "Binary Point 'b'"; n_bits_ab "Number of Bits 'ab'"; bin_pt_ab "Binary Point 'ab'"; in_latency "Input latency"; mult_latency "Multiplier Latency"; add_latency "Adder Latency"; conv_latency "Convert latency"; conjugated "Conjugate"; async "asynchronous operation"; pipelined_enable "enable pipeline"; multiplier_implementation "Multiplier implementation"
      mask help:
      | Multiplies two complex numbers using 4 multipliers and 2 adders.
      | Conjugation is optional.
      mask init: same as s_b16a4x32kf/sys0/xeng/auto_tap/dual_pol_cmac/cmac/cmult*
      settings: AttributesFormatString=|
      | 8_7 * 8_7 ==> 25_14
      | Truncate, Wrap
      | Latency=0
      mask TypeOptions quantization: Truncate | Round  (unbiased: +/- Inf) | Round  (unbiased: Even Values)
      mask TypeOptions overflow: Wrap | Saturate | Flag as error
      mask TypeOptions multiplier_implementation: behavioral HDL | standard core | embedded multiplier core
  ri_to_c : Subsystem
  acc_out : Outport
  valid_out : Outport  Port=2
  wires:
  cmult*/1(ab) -> c_to_ri1/1(In1)
  valid_in/1 -> acc1/4(valid_in)
  acc1/2(valid_out) -> valid_out/1
  acc/2(valid_out) -> Terminator/1
  Constant2/1 -> acc/4(valid_in)
  Delay/1 -> Counter/1
  sync/1 -> Delay/1
  Constant1/1 -> Relational/2
  Counter/1 -> Relational/1
  Relational/1 -> acc1/1(rst), acc/1(rst)
  c_to_ri2/2(Out2) -> acc1/3(acc_in)
  ri_to_c/1(Out1) -> acc_out/1
  acc1/1(acc_out) -> ri_to_c/2(In2)
  acc_in/1 -> c_to_ri2/1(In1)
  c+di/1 -> cmult*/2(b)
  a+bi/1 -> cmult*/1(a)
  c_to_ri1/1(Out1) -> acc/2(din)  "auto_real"
  c_to_ri1/2(Out2) -> acc1/2(din)
  acc/1(acc_out) -> ri_to_c/1(In1)
  c_to_ri2/1(Out1) -> acc/3(acc_in)

== system s_b16a4x32kf/sys3/xeng/baseline_tap4/dual_pol_cmac/cmac1 ==
  a+bi : Inport
  c+di : Inport  Port=2
  acc_in : Inport  Port=3
  sync : Inport  Port=4
  valid_in : Inport  Port=5
  Constant1 : xbsIndex_r4/Constant  const=0  gui_display_data_type=Fixed-point  arith_type=Unsigned  n_bits=bit_growth  bin_pt=0  preci_type=Single  exp_width=8  frac_width=24  explicit_period=on  period=1  equ=P=C  opselect=C  inp2=PCIN>>17  opr=+  inp1=P  carry=CIN  dbl_ovrd=off  block_type=constant
      settings: block_version=9.2.01
  Constant2 : xbsIndex_r4/Constant  const=0  gui_display_data_type=Fixed-point  arith_type=Unsigned  n_bits=1  bin_pt=0  preci_type=Single  exp_width=8  frac_width=24  explicit_period=off  period=1  equ=P=C  opselect=C  inp2=PCIN>>17  opr=+  inp1=P  carry=CIN  dbl_ovrd=off  block_type=constant
      settings: block_version=9.2.01
  Counter : xbsIndex_r4/Counter  cnt_type=Count Limited  cnt_to=acc_len - 1  operation=Up  start_count=0  cnt_by_val=1  arith_type=Unsigned  n_bits=bit_growth  bin_pt=0  load_pin=off  rst=on  en=off  explicit_period=off  period=1  use_behavioral_HDL=off  implementation=Fabric  use_rpm=on  dbl_ovrd=off  block_type=counter
      settings: xl_area=[0, 0, 0, 0, 0, 0, 0]  block_version=9.2.01
  Delay : xbsIndex_r4/Delay  rst=off  infoeditControl=Selection of Reset will increase slice count due to use of real FFs and instead of SRLs  en=off  latency=add_latency + mult_latency - 1  reg_retiming=on  dbl_ovrd=off  block_type=delay
      settings: xl_area=[0, 0, 0, 0, 0, 0, 0]  block_version=9.2.01
  Relational : xbsIndex_r4/Relational  mode=a=b  op_type=Bool  en=off  latency=1  dbl_ovrd=off  block_type=relational
      settings: xl_area=[0, 0, 0, 0, 0, 0, 0]  block_version=9.2.01
  Terminator : Terminator
  acc : Subsystem
  acc1 : Subsystem
  c_to_ri1 : Subsystem
  c_to_ri2 : Subsystem
  cmult* : Subsystem  AncestorBlock=casper_library_multipliers/cmult  mask(cmult){n_bits_a=8, bin_pt_a=7, n_bits_b=8, bin_pt_b=7, n_bits_ab=25, bin_pt_ab=14, quantization=Truncate, overflow=Wrap, in_latency=0, mult_latency=4, add_latency=3, conv_latency=0, conjugated=on, async=off, pipelined_enable=on, multiplier_implementation=embedded multiplier core}
      mask prompts: n_bits_a "Number of Bits 'a'"; bin_pt_a "Binary Point 'a'"; n_bits_b "Number of Bits 'b'"; bin_pt_b "Binary Point 'b'"; n_bits_ab "Number of Bits 'ab'"; bin_pt_ab "Binary Point 'ab'"; in_latency "Input latency"; mult_latency "Multiplier Latency"; add_latency "Adder Latency"; conv_latency "Convert latency"; conjugated "Conjugate"; async "asynchronous operation"; pipelined_enable "enable pipeline"; multiplier_implementation "Multiplier implementation"
      mask help:
      | Multiplies two complex numbers using 4 multipliers and 2 adders.
      | Conjugation is optional.
      mask init: same as s_b16a4x32kf/sys0/xeng/auto_tap/dual_pol_cmac/cmac/cmult*
      settings: AttributesFormatString=|
      | 8_7 * 8_7 ==> 25_14
      | Truncate, Wrap
      | Latency=0
      mask TypeOptions quantization: Truncate | Round  (unbiased: +/- Inf) | Round  (unbiased: Even Values)
      mask TypeOptions overflow: Wrap | Saturate | Flag as error
      mask TypeOptions multiplier_implementation: behavioral HDL | standard core | embedded multiplier core
  ri_to_c : Subsystem
  acc_out : Outport
  valid_out : Outport  Port=2
  wires:
  cmult*/1(ab) -> c_to_ri1/1(In1)
  valid_in/1 -> acc1/4(valid_in)
  acc1/2(valid_out) -> valid_out/1
  acc/2(valid_out) -> Terminator/1
  Constant2/1 -> acc/4(valid_in)
  Delay/1 -> Counter/1
  sync/1 -> Delay/1
  Constant1/1 -> Relational/2
  Counter/1 -> Relational/1
  Relational/1 -> acc1/1(rst), acc/1(rst)
  c_to_ri2/2(Out2) -> acc1/3(acc_in)
  ri_to_c/1(Out1) -> acc_out/1
  acc1/1(acc_out) -> ri_to_c/2(In2)
  acc_in/1 -> c_to_ri2/1(In1)
  c+di/1 -> cmult*/2(b)
  a+bi/1 -> cmult*/1(a)
  c_to_ri1/1(Out1) -> acc/2(din)  "auto_real"
  c_to_ri1/2(Out2) -> acc1/2(din)
  acc/1(acc_out) -> ri_to_c/1(In1)
  c_to_ri2/1(Out1) -> acc/3(acc_in)

== system s_b16a4x32kf/sys3/xeng/baseline_tap4/dual_pol_cmac/cmac2 ==
  a+bi : Inport
  c+di : Inport  Port=2
  acc_in : Inport  Port=3
  sync : Inport  Port=4
  valid_in : Inport  Port=5
  Constant1 : xbsIndex_r4/Constant  const=0  gui_display_data_type=Fixed-point  arith_type=Unsigned  n_bits=bit_growth  bin_pt=0  preci_type=Single  exp_width=8  frac_width=24  explicit_period=on  period=1  equ=P=C  opselect=C  inp2=PCIN>>17  opr=+  inp1=P  carry=CIN  dbl_ovrd=off  block_type=constant
      settings: block_version=9.2.01
  Constant2 : xbsIndex_r4/Constant  const=0  gui_display_data_type=Fixed-point  arith_type=Unsigned  n_bits=1  bin_pt=0  preci_type=Single  exp_width=8  frac_width=24  explicit_period=off  period=1  equ=P=C  opselect=C  inp2=PCIN>>17  opr=+  inp1=P  carry=CIN  dbl_ovrd=off  block_type=constant
      settings: block_version=9.2.01
  Counter : xbsIndex_r4/Counter  cnt_type=Count Limited  cnt_to=acc_len - 1  operation=Up  start_count=0  cnt_by_val=1  arith_type=Unsigned  n_bits=bit_growth  bin_pt=0  load_pin=off  rst=on  en=off  explicit_period=off  period=1  use_behavioral_HDL=off  implementation=Fabric  use_rpm=on  dbl_ovrd=off  block_type=counter
      settings: xl_area=[0, 0, 0, 0, 0, 0, 0]  block_version=9.2.01
  Delay : xbsIndex_r4/Delay  rst=off  infoeditControl=Selection of Reset will increase slice count due to use of real FFs and instead of SRLs  en=off  latency=add_latency + mult_latency - 1  reg_retiming=on  dbl_ovrd=off  block_type=delay
      settings: xl_area=[0, 0, 0, 0, 0, 0, 0]  block_version=9.2.01
  Relational : xbsIndex_r4/Relational  mode=a=b  op_type=Bool  en=off  latency=1  dbl_ovrd=off  block_type=relational
      settings: xl_area=[0, 0, 0, 0, 0, 0, 0]  block_version=9.2.01
  Terminator : Terminator
  acc : Subsystem
  acc1 : Subsystem
  c_to_ri1 : Subsystem
  c_to_ri2 : Subsystem
  cmult* : Subsystem  AncestorBlock=casper_library_multipliers/cmult  mask(cmult){n_bits_a=8, bin_pt_a=7, n_bits_b=8, bin_pt_b=7, n_bits_ab=25, bin_pt_ab=14, quantization=Truncate, overflow=Wrap, in_latency=0, mult_latency=4, add_latency=3, conv_latency=0, conjugated=on, async=off, pipelined_enable=on, multiplier_implementation=embedded multiplier core}
      mask prompts: n_bits_a "Number of Bits 'a'"; bin_pt_a "Binary Point 'a'"; n_bits_b "Number of Bits 'b'"; bin_pt_b "Binary Point 'b'"; n_bits_ab "Number of Bits 'ab'"; bin_pt_ab "Binary Point 'ab'"; in_latency "Input latency"; mult_latency "Multiplier Latency"; add_latency "Adder Latency"; conv_latency "Convert latency"; conjugated "Conjugate"; async "asynchronous operation"; pipelined_enable "enable pipeline"; multiplier_implementation "Multiplier implementation"
      mask help:
      | Multiplies two complex numbers using 4 multipliers and 2 adders.
      | Conjugation is optional.
      mask init: same as s_b16a4x32kf/sys0/xeng/auto_tap/dual_pol_cmac/cmac/cmult*
      settings: AttributesFormatString=|
      | 8_7 * 8_7 ==> 25_14
      | Truncate, Wrap
      | Latency=0
      mask TypeOptions quantization: Truncate | Round  (unbiased: +/- Inf) | Round  (unbiased: Even Values)
      mask TypeOptions overflow: Wrap | Saturate | Flag as error
      mask TypeOptions multiplier_implementation: behavioral HDL | standard core | embedded multiplier core
  ri_to_c : Subsystem
  acc_out : Outport
  valid_out : Outport  Port=2
  wires:
  cmult*/1(ab) -> c_to_ri1/1(In1)
  valid_in/1 -> acc1/4(valid_in)
  acc1/2(valid_out) -> valid_out/1
  acc/2(valid_out) -> Terminator/1
  Constant2/1 -> acc/4(valid_in)
  Delay/1 -> Counter/1
  sync/1 -> Delay/1
  Constant1/1 -> Relational/2
  Counter/1 -> Relational/1
  Relational/1 -> acc1/1(rst), acc/1(rst)
  c_to_ri2/2(Out2) -> acc1/3(acc_in)
  ri_to_c/1(Out1) -> acc_out/1
  acc1/1(acc_out) -> ri_to_c/2(In2)
  acc_in/1 -> c_to_ri2/1(In1)
  c+di/1 -> cmult*/2(b)
  a+bi/1 -> cmult*/1(a)
  c_to_ri1/1(Out1) -> acc/2(din)  "auto_real"
  c_to_ri1/2(Out2) -> acc1/2(din)
  acc/1(acc_out) -> ri_to_c/1(In1)
  c_to_ri2/1(Out1) -> acc/3(acc_in)

== system s_b16a4x32kf/sys3/xeng/baseline_tap4/dual_pol_cmac/cmac3 ==
  a+bi : Inport
  c+di : Inport  Port=2
  acc_in : Inport  Port=3
  sync : Inport  Port=4
  valid_in : Inport  Port=5
  Constant1 : xbsIndex_r4/Constant  const=0  gui_display_data_type=Fixed-point  arith_type=Unsigned  n_bits=bit_growth  bin_pt=0  preci_type=Single  exp_width=8  frac_width=24  explicit_period=on  period=1  equ=P=C  opselect=C  inp2=PCIN>>17  opr=+  inp1=P  carry=CIN  dbl_ovrd=off  block_type=constant
      settings: block_version=9.2.01
  Constant2 : xbsIndex_r4/Constant  const=0  gui_display_data_type=Fixed-point  arith_type=Unsigned  n_bits=1  bin_pt=0  preci_type=Single  exp_width=8  frac_width=24  explicit_period=off  period=1  equ=P=C  opselect=C  inp2=PCIN>>17  opr=+  inp1=P  carry=CIN  dbl_ovrd=off  block_type=constant
      settings: block_version=9.2.01
  Counter : xbsIndex_r4/Counter  cnt_type=Count Limited  cnt_to=acc_len - 1  operation=Up  start_count=0  cnt_by_val=1  arith_type=Unsigned  n_bits=bit_growth  bin_pt=0  load_pin=off  rst=on  en=off  explicit_period=off  period=1  use_behavioral_HDL=off  implementation=Fabric  use_rpm=on  dbl_ovrd=off  block_type=counter
      settings: xl_area=[0, 0, 0, 0, 0, 0, 0]  block_version=9.2.01
  Delay : xbsIndex_r4/Delay  rst=off  infoeditControl=Selection of Reset will increase slice count due to use of real FFs and instead of SRLs  en=off  latency=add_latency + mult_latency - 1  reg_retiming=on  dbl_ovrd=off  block_type=delay
      settings: xl_area=[0, 0, 0, 0, 0, 0, 0]  block_version=9.2.01
  Relational : xbsIndex_r4/Relational  mode=a=b  op_type=Bool  en=off  latency=1  dbl_ovrd=off  block_type=relational
      settings: xl_area=[0, 0, 0, 0, 0, 0, 0]  block_version=9.2.01
  Terminator : Terminator
  acc : Subsystem
  acc1 : Subsystem
  c_to_ri1 : Subsystem
  c_to_ri2 : Subsystem
  cmult* : Subsystem  AncestorBlock=casper_library_multipliers/cmult  mask(cmult){n_bits_a=8, bin_pt_a=7, n_bits_b=8, bin_pt_b=7, n_bits_ab=25, bin_pt_ab=14, quantization=Truncate, overflow=Wrap, in_latency=0, mult_latency=4, add_latency=3, conv_latency=0, conjugated=on, async=off, pipelined_enable=on, multiplier_implementation=embedded multiplier core}
      mask prompts: n_bits_a "Number of Bits 'a'"; bin_pt_a "Binary Point 'a'"; n_bits_b "Number of Bits 'b'"; bin_pt_b "Binary Point 'b'"; n_bits_ab "Number of Bits 'ab'"; bin_pt_ab "Binary Point 'ab'"; in_latency "Input latency"; mult_latency "Multiplier Latency"; add_latency "Adder Latency"; conv_latency "Convert latency"; conjugated "Conjugate"; async "asynchronous operation"; pipelined_enable "enable pipeline"; multiplier_implementation "Multiplier implementation"
      mask help:
      | Multiplies two complex numbers using 4 multipliers and 2 adders.
      | Conjugation is optional.
      mask init: same as s_b16a4x32kf/sys0/xeng/auto_tap/dual_pol_cmac/cmac/cmult*
      settings: AttributesFormatString=|
      | 8_7 * 8_7 ==> 25_14
      | Truncate, Wrap
      | Latency=0
      mask TypeOptions quantization: Truncate | Round  (unbiased: +/- Inf) | Round  (unbiased: Even Values)
      mask TypeOptions overflow: Wrap | Saturate | Flag as error
      mask TypeOptions multiplier_implementation: behavioral HDL | standard core | embedded multiplier core
  ri_to_c : Subsystem
  acc_out : Outport
  valid_out : Outport  Port=2
  wires:
  cmult*/1(ab) -> c_to_ri1/1(In1)
  valid_in/1 -> acc1/4(valid_in)
  acc1/2(valid_out) -> valid_out/1
  acc/2(valid_out) -> Terminator/1
  Constant2/1 -> acc/4(valid_in)
  Delay/1 -> Counter/1
  sync/1 -> Delay/1
  Constant1/1 -> Relational/2
  Counter/1 -> Relational/1
  Relational/1 -> acc1/1(rst), acc/1(rst)
  c_to_ri2/2(Out2) -> acc1/3(acc_in)
  ri_to_c/1(Out1) -> acc_out/1
  acc1/1(acc_out) -> ri_to_c/2(In2)
  acc_in/1 -> c_to_ri2/1(In1)
  c+di/1 -> cmult*/2(b)
  a+bi/1 -> cmult*/1(a)
  c_to_ri1/1(Out1) -> acc/2(din)  "auto_real"
  c_to_ri1/2(Out2) -> acc1/2(din)
  acc/1(acc_out) -> ri_to_c/1(In1)
  c_to_ri2/1(Out1) -> acc/3(acc_in)
